simulink library "Lib_Piccolo"  (R2018b)
settings: Solver=VariableStepAuto  StartTime=0.0  StopTime=10.0  RelTol=1e-3
values from neighbouring files (symbols this model uses):
  AccelErrInt2Brakes = 0.15    [SimulationControlConfig16P.m]    (also in SimulationControlConfig16P_LEGACY.m; SimulationControlConfigTAILLESS.m = 0.2; SimulationControlConfigUTAIL.m = 0.2)
  AileronMax = 25    [SimulationControlConfig16P.m]    (also in SimulationControlConfig16P_LEGACY.m; SimulationControlConfigTAILLESS.m; SimulationControlConfigUTAIL.m)
  AileronPower = 0.00268    [SimulationControlConfig16P.m]    (also in SimulationControlConfig16P_LEGACY.m; SimulationControlConfigTAILLESS.m; SimulationControlConfigUTAIL.m)
  AileronSurfaceMax = 45    [SimulationControlConfig16P.m]    (also in SimulationControlConfig16P_LEGACY.m)
  AileronTrim = 0    [SimulationControlConfig16P.m]    (also in SimulationControlConfig16P_LEGACY.m; SimulationControlConfigTAILLESS.m; SimulationControlConfigUTAIL.m)
  Alt = 1000 + TerrainHeight    [SimulationStateConfig.m]
  AltCruise_m = testPlans(testIndx).terrainElevation * 0.3048 + 200    [SimulationControlConfig16P.m]    (also in SimulationControlConfigTAILLESS.m = 1083; SimulationControlConfigUTAIL.m = testPlans(testIndx).terrainElevation * 0.3048 + 152)
  AltitudeRate2PitchCmdIntegratorInit = 0.1    [SimulationControlPre.m]
  AltMax = 10000    [SimulationControlConfig16P.m]    (also in SimulationControlConfig16P_LEGACY.m; SimulationControlConfigTAILLESS.m; SimulationControlConfigUTAIL.m)
  AltMaxAccel = 1.25    [SimulationControlConfig16P.m]    (also in SimulationControlConfig16P_LEGACY.m = 0.9; SimulationControlConfigTAILLESS.m = 1.7; SimulationControlConfigUTAIL.m = 2)
  AltMin = 0    [SimulationControlConfig16P.m]    (also in SimulationControlConfig16P_LEGACY.m; SimulationControlConfigTAILLESS.m; SimulationControlConfigUTAIL.m)
  AltRateCmd2Pitch = 0.50    (= 0.5)    [SimulationControlConfig16P.m]    (also in SimulationControlConfig16P_LEGACY.m = 0.6; SimulationControlConfigTAILLESS.m = 0.2; SimulationControlConfigUTAIL.m = 0.3)
  AltRateError2Pitch = 0.40    (= 0.4)    [SimulationControlConfig16P.m]    (also in SimulationControlConfig16P_LEGACY.m; SimulationControlConfigTAILLESS.m = 0.55; SimulationControlConfigUTAIL.m = 0.55)
  AltRateErrorInt2Pitch = 0.50    (= 0.5)    [SimulationControlConfig16P.m]    (also in SimulationControlConfig16P_LEGACY.m = 0.45; SimulationControlConfigTAILLESS.m; SimulationControlConfigUTAIL.m = 0.75)
  AltRateLpfCutOff = 3    [SimulationControlConfig16P.m]    (also in SimulationControlConfig16P_LEGACY.m; SimulationControlConfigTAILLESS.m = 2; SimulationControlConfigUTAIL.m = 2)
  AutoNosegear2Rudder = 26    [SimulationControlConfig16P.m]    (also in SimulationControlConfig16P_LEGACY.m; SimulationControlConfigTAILLESS.m = 25.2; SimulationControlConfigUTAIL.m = 14)
  b = 5.54    [SimulationControlConfig16P.m]    (also in SimulationControlConfig16P_LEGACY.m; SimulationControlConfigTAILLESS.m = 2.37; SimulationControlConfigUTAIL.m = 2.37)
  Bank2AileronIntegratorInit = 0    [SimulationControlPre.m]
  BankMax_User = BankMax_User/180*pi    (= 0.523598775598)    [SimulationControlConfig16P.m]    (also in SimulationControlConfig16P_LEGACY.m; SimulationControlConfigTAILLESS.m = 0.610865238198; SimulationControlConfigUTAIL.m = 0.628318530718)
  baseLegFlaps = 20    [SimulationControlConfig16P.m]    (also in SimulationControlConfig16P_LEGACY.m = 0; SimulationControlConfigTAILLESS.m = 15; SimulationControlConfigUTAIL.m = 10)
  C = GeneticOpt.C    [SimulationCostFunction.m]
  c = Sw/b    (= 0.841696750903)    [SimulationControlConfig16P.m]    (also in SimulationControlConfig16P_LEGACY.m; SimulationControlConfigTAILLESS.m = 0.354008438819; SimulationControlConfigUTAIL.m = 0.354008438819)
  cell2WheelFactorMG = 5.98    [SimulationSensorConfig16P_LEGACY.m]
  cell2WheelFactorNG = 1    [SimulationSensorConfig16P_LEGACY.m]
  cellSatMaxMG = 15000    [SimulationSensorConfig16P.m]    (also in SimulationSensorConfig16P_LEGACY.m; SimulationSensorConfigTAILLESS7P.m; SimulationSensorConfigUTAIL7P.m)
  cellSatMaxNG = 1000    [SimulationSensorConfig16P.m]    (also in SimulationSensorConfig16P_LEGACY.m; SimulationSensorConfigTAILLESS7P.m; SimulationSensorConfigUTAIL7P.m)
  cellSatMinMG = -15000    [SimulationSensorConfig16P.m]    (also in SimulationSensorConfig16P_LEGACY.m; SimulationSensorConfigTAILLESS7P.m; SimulationSensorConfigUTAIL7P.m)
  cellSatMinNG = -1000    [SimulationSensorConfig16P.m]    (also in SimulationSensorConfig16P_LEGACY.m; SimulationSensorConfigTAILLESS7P.m; SimulationSensorConfigUTAIL7P.m)
  CL_Limit = CL_Max    (= 0.54)    [SimulationControlConfig16P.m]    (also in SimulationControlConfig16P_LEGACY.m; SimulationControlConfigTAILLESS.m; SimulationControlConfigUTAIL.m = 0.53)
  CL_Max = 0.54    [SimulationControlConfig16P.m]    (also in SimulationControlConfig16P_LEGACY.m; SimulationControlConfigTAILLESS.m; SimulationControlConfigUTAIL.m = 0.53)
  CL_Max_Nom = 0.465    [SimulationControlConfig16P.m]    (also in SimulationControlConfig16P_LEGACY.m; SimulationControlConfigTAILLESS.m = 0.39; SimulationControlConfigUTAIL.m)
  CL_Min = 0    [SimulationControlConfig16P.m]    (also in SimulationControlConfig16P_LEGACY.m; SimulationControlConfigTAILLESS.m; SimulationControlConfigUTAIL.m)
  ClimbMaxFraction = 0.35    [SimulationControlConfig16P.m]    (also in SimulationControlConfig16P_LEGACY.m = 0.24; SimulationControlConfigTAILLESS.m = 0.19; SimulationControlConfigUTAIL.m = 0.21)
  ClimboutMaxBank = 7.0    (= 7)    [SimulationControlConfig16P.m]    (also in SimulationControlConfig16P_LEGACY.m; SimulationControlConfigTAILLESS.m = 5; SimulationControlConfigUTAIL.m)
  ClimboutTimer = 7.0    (= 7)    [SimulationControlConfig16P.m]    (also in SimulationControlConfig16P_LEGACY.m; SimulationControlConfigTAILLESS.m; SimulationControlConfigUTAIL.m)
  dCl_per_dFlap = 0.005581818    [SimulationControlConfig16P.m]    (also in SimulationControlConfig16P_LEGACY.m = 0; SimulationControlConfigTAILLESS.m = 0; SimulationControlConfigUTAIL.m = 0)
  DecelerationCmd = 3.1    [SimulationControlConfig16P.m]    (also in SimulationControlConfig16P_LEGACY.m; SimulationControlConfigTAILLESS.m = 0.1; SimulationControlConfigUTAIL.m = 0.1)
  DeRotateLogicEndTimer = abs((NoseDownLimit_Deg-1)/DeRotateRamp_Dps)    [SimulationControlConfig16P.m]    (also in SimulationControlConfig16P_LEGACY.m; SimulationControlConfigTAILLESS.m; SimulationControlConfigUTAIL.m)
  DeRotateLogicHoldNoseUpTimer = 0.1    [SimulationControlConfig16P.m]    (also in SimulationControlConfig16P_LEGACY.m; SimulationControlConfigTAILLESS.m; SimulationControlConfigUTAIL.m)
  DeRotateLogicTimerTimeout = 2    [SimulationControlConfig16P.m]    (also in SimulationControlConfig16P_LEGACY.m; SimulationControlConfigTAILLESS.m; SimulationControlConfigUTAIL.m)
  DeRotateLowerCmdSaturation = 0    [SimulationControlConfig16P.m]    (also in SimulationControlConfig16P_LEGACY.m; SimulationControlConfigTAILLESS.m; SimulationControlConfigUTAIL.m)
  DeRotateRamp_Dps = 3    [SimulationControlConfig16P.m]    (also in SimulationControlConfig16P_LEGACY.m; SimulationControlConfigTAILLESS.m = 8; SimulationControlConfigUTAIL.m = 8)
  DeRotateUpperCmdSaturation = 7    [SimulationControlConfig16P.m]    (also in SimulationControlConfig16P_LEGACY.m; SimulationControlConfigTAILLESS.m; SimulationControlConfigUTAIL.m)
  DescentMaxFraction = 0.22    [SimulationControlConfig16P.m]    (also in SimulationControlConfig16P_LEGACY.m = 0.2; SimulationControlConfigTAILLESS.m = 0.17; SimulationControlConfigUTAIL.m = 0.17)
  DesktopSimTerrainOffset_m = 0.406    [SimulationAircraftConfig.m]
  downwindFlaps = 0    [SimulationControlConfig16P.m]    (also in SimulationControlConfig16P_LEGACY.m; SimulationControlConfigTAILLESS.m; SimulationControlConfigUTAIL.m)
  DP_init = 0.5*1.225*V_init^2    [SimulationControlConfig16P.m]    (also in SimulationControlConfig16P_LEGACY.m; SimulationControlConfigTAILLESS.m; SimulationControlConfigUTAIL.m)
  dscNoiseMG = 1    [SimulationSensorConfig16P_LEGACY.m]
  dscNoiseNG = 0.25    [SimulationSensorConfig16P_LEGACY.m]
  DSCnumBits = 24    [SimulationSensorConfig16P.m]    (also in SimulationSensorConfig16P_LEGACY.m; SimulationSensorConfigTAILLESS7P.m; SimulationSensorConfigUTAIL7P.m)
  DSCRangeMaxMG = 15000    [SimulationSensorConfig16P.m]    (also in SimulationSensorConfig16P_LEGACY.m; SimulationSensorConfigTAILLESS7P.m; SimulationSensorConfigUTAIL7P.m)
  DSCRangeMaxNG = 1000    [SimulationSensorConfig16P.m]    (also in SimulationSensorConfig16P_LEGACY.m; SimulationSensorConfigTAILLESS7P.m; SimulationSensorConfigUTAIL7P.m)
  DSCRangeMinMG = -15000    [SimulationSensorConfig16P.m]    (also in SimulationSensorConfig16P_LEGACY.m; SimulationSensorConfigTAILLESS7P.m; SimulationSensorConfigUTAIL7P.m)
  DSCRangeMinNG = -1000    [SimulationSensorConfig16P.m]    (also in SimulationSensorConfig16P_LEGACY.m; SimulationSensorConfigTAILLESS7P.m; SimulationSensorConfigUTAIL7P.m)
  dt = DLLSim.dt    [SimulationTimeStep.m]    (also in SimulationTrim.m = 0.02)
  EarlyTouchdownThreshold = 3.0    (= 3)    [SimulationControlConfig16P.m]    (also in SimulationControlConfig16P_LEGACY.m; SimulationControlConfigTAILLESS.m = 2.2; SimulationControlConfigUTAIL.m = 2.5)
  ElevatorDeflectionRate = 15    [SimulationControlConfig16P.m]    (also in SimulationControlConfig16P_LEGACY.m = 12; SimulationControlConfigTAILLESS.m = 10; SimulationControlConfigUTAIL.m = 12)
  ElevatorMax = 25    [SimulationControlConfig16P.m]    (also in SimulationControlConfig16P_LEGACY.m; SimulationControlConfigTAILLESS.m; SimulationControlConfigUTAIL.m)
  ElevatorPower = -0.002209    [SimulationControlConfig16P.m]    (also in SimulationControlConfig16P_LEGACY.m; SimulationControlConfigTAILLESS.m = -0.002956; SimulationControlConfigUTAIL.m = -0.00205983)
  ElevatorTrim = -3.5    [SimulationControlConfig16P.m]    (also in SimulationControlConfig16P_LEGACY.m; SimulationControlConfigTAILLESS.m = -6; SimulationControlConfigUTAIL.m = -8)
  elevonBias = 0    [SimulationControlConfig16P.m]    (also in SimulationControlConfig16P_LEGACY.m; SimulationControlConfigTAILLESS.m; SimulationControlConfigUTAIL.m)
  Enable_TAS_Protection = 0    [SimulationControlConfig16P.m]    (also in SimulationControlConfig16P_LEGACY.m; SimulationControlConfigTAILLESS.m; SimulationControlConfigUTAIL.m)
  EnableCrossTrackAbort = 1    [SimulationControlConfig16P.m]    (also in SimulationControlConfigTAILLESS.m; SimulationControlConfigUTAIL.m)
  EnergyBandwidth = 0.02    [SimulationControlConfig16P.m]    (also in SimulationControlConfig16P_LEGACY.m; SimulationControlConfigTAILLESS.m = 0.06; SimulationControlConfigUTAIL.m = 0.06)
  EngineLhFuelCut = 0    [SimulationAircraftConfig.m]
  EngineRhFuelCut = 0    [SimulationAircraftConfig.m]
  FastThrottleRate = 0.075    [SimulationControlConfig16P.m]    (also in SimulationControlConfig16P_LEGACY.m = 0.05; SimulationControlConfigTAILLESS.m = 0.1; SimulationControlConfigUTAIL.m = 0.1)
  FilterWarmUpTime = 2    [SimulationSensorConfig16P.m]    (also in SimulationSensorConfig16P_LEGACY.m; SimulationSensorConfigTAILLESS7P.m; SimulationSensorConfigUTAIL7P.m)
  finalApproachFlaps = 20    [SimulationControlConfig16P.m]    (also in SimulationControlConfig16P_LEGACY.m = 0; SimulationControlConfigTAILLESS.m = 22; SimulationControlConfigUTAIL.m = 10)
  FinalDescentSlope_Deg = testPlans(testIndx).descentSlope    [SimulationControlConfig16P.m]    (also in SimulationControlConfig16P_LEGACY.m; SimulationControlConfigTAILLESS.m; SimulationControlConfigUTAIL.m)
  flapMax = 0    [SimulationControlConfig16P.m]    (also in SimulationControlConfig16P_LEGACY.m; SimulationControlConfigTAILLESS.m; SimulationControlConfigUTAIL.m)
  flapRate = 7.5    [SimulationControlConfig16P.m]    (also in SimulationControlConfig16P_LEGACY.m; SimulationControlConfigTAILLESS.m = 6.6; SimulationControlConfigUTAIL.m)
  FlareHeight = 5    [SimulationControlConfig16P.m]    (also in SimulationControlConfig16P_LEGACY.m = 4.8; SimulationControlConfigTAILLESS.m = 2.5; SimulationControlConfigUTAIL.m = 2)
  FlareVerticalRate_mps = -0.4    [SimulationControlConfig16P.m]    (also in SimulationControlConfig16P_LEGACY.m = -0.5; SimulationControlConfigTAILLESS.m = -0.15; SimulationControlConfigUTAIL.m = -0.15)
  Fp_Aileron = 0.55*2*pi*RollRateLpfCutoff*dt    [SimulationControlConfig16P.m]    (also in SimulationControlConfig16P_LEGACY.m; SimulationControlConfigTAILLESS.m; SimulationControlConfigUTAIL.m)
  Fp_Alt = 0.55*AltBandwidth    (= 0.099)    [SimulationControlConfig16P.m]    (also in SimulationControlConfig16P_LEGACY.m; SimulationControlConfigTAILLESS.m = 0.587477826221; SimulationControlConfigUTAIL.m = 0.69115038379)
  Fp_AltRate = 0.55*2*pi*AltRateLpfCutOff*dt    [SimulationControlConfig16P.m]    (also in SimulationControlConfig16P_LEGACY.m; SimulationControlConfigTAILLESS.m; SimulationControlConfigUTAIL.m)
  Fp_Elevator = 0.55*2*pi*PitchRateLpfCutoff*dt    [SimulationControlConfig16P.m]    (also in SimulationControlConfig16P_LEGACY.m; SimulationControlConfigTAILLESS.m; SimulationControlConfigUTAIL.m)
  Fp_Energy = 0.55*2*pi*EnergyBandwidth    (= 0.069115038379)    [SimulationControlConfig16P.m]    (also in SimulationControlConfig16P_LEGACY.m; SimulationControlConfigTAILLESS.m = 0.207345115137; SimulationControlConfigUTAIL.m = 0.207345115137)
  Fp_Energy2 = 0.55*2*pi*EnergyBandwidth*dt    [SimulationControlConfig16P.m]    (also in SimulationControlConfig16P_LEGACY.m; SimulationControlConfigTAILLESS.m; SimulationControlConfigUTAIL.m)
  Fp_Pitch = 0.55*2*pi*PitchBandwidth    (= 2.76460153516)    [SimulationControlConfig16P.m]    (also in SimulationControlConfig16P_LEGACY.m = 3.11017672705; SimulationControlConfigTAILLESS.m = 3.80132711084; SimulationControlConfigUTAIL.m = 2.41902634326)
  Fp_Pitch_2 = 0.55*2*pi*PitchBandwidth*dt    [SimulationControlConfig16P.m]    (also in SimulationControlConfig16P_LEGACY.m; SimulationControlConfigTAILLESS.m; SimulationControlConfigUTAIL.m)
  Fp_Roll = RollBandwidth^2    (= 1)    [SimulationControlConfig16P.m]    (also in SimulationControlConfig16P_LEGACY.m = 1.44; SimulationControlConfigTAILLESS.m; SimulationControlConfigUTAIL.m)
  Fp_Rudder = 0.55*2*pi*YawRateLpfCutoff*dt    [SimulationControlConfig16P.m]    (also in SimulationControlConfig16P_LEGACY.m; SimulationControlConfigTAILLESS.m; SimulationControlConfigUTAIL.m)
  Fp_TAS = 0.55*2*pi*TASBandwidth    (= 0.103672557568)    [SimulationControlConfig16P.m]    (also in SimulationControlConfig16P_LEGACY.m; SimulationControlConfigTAILLESS.m = 0.172787595947; SimulationControlConfigUTAIL.m = 0.172787595947)
  Fp_TAS_Filter = 2*pi*TasLpfCutoff*dt    [SimulationControlConfig16P.m]    (also in SimulationControlConfig16P_LEGACY.m; SimulationControlConfigTAILLESS.m; SimulationControlConfigUTAIL.m)
  Fp_Turn = 0.55*2*pi*TurnErrLPFcutoff    (= 0.0345575191895)    [SimulationControlConfig16P.m]    (also in SimulationControlConfig16P_LEGACY.m; SimulationControlConfigTAILLESS.m = 0.172787595947; SimulationControlConfigUTAIL.m = 0.172787595947)
  Fp_TurnDerr = 0.55*2*pi*TurnDerivativeLPFcutoff    (= 0.0345575191895)    [SimulationControlConfig16P.m]    (also in SimulationControlConfig16P_LEGACY.m; SimulationControlConfigTAILLESS.m = 0.172787595947; SimulationControlConfigUTAIL.m = 0.172787595947)
  FTV = 3    [SimulationAircraftConfig.m]
  ftvStaticPositionError = 1/1.18    (= 0.847457627119)    [SimulationSensorConfig16P.m]    (also in SimulationSensorConfig16P_LEGACY.m; SimulationSensorConfigTAILLESS7P.m = 1; SimulationSensorConfigUTAIL7P.m = 1)
  g = 9.81    [SimulationStateConfig.m]
  GustSpd_Kts = testPlans(testIndx).gustSpd    [SimulationStateConfig.m]
  GustTriggerVal = testPlans(testIndx).gustTriggerVal    [SimulationStateConfig.m]
  HeadingErr2TurnRate = 0.5    [SimulationControlConfig16P.m]    (also in SimulationControlConfig16P_LEGACY.m; SimulationControlConfigTAILLESS.m; SimulationControlConfigUTAIL.m)
  HeadingErrDer2TurnRate = 0.3    [SimulationControlConfig16P.m]    (also in SimulationControlConfig16P_LEGACY.m; SimulationControlConfigTAILLESS.m; SimulationControlConfigUTAIL.m)
  IASbounce = IASstall*0.8    [SimulationControlPre.m]
  IAScruiseCMD = sqrt(2*m*9.81/(1.225*Sw*CL_cruise))    [SimulationControlConfig16P.m]    (also in SimulationControlConfig16P_LEGACY.m; SimulationControlConfigTAILLESS.m; SimulationControlConfigUTAIL.m)
  IASfinalCMD = 1.12 * IASmin    [SimulationControlConfig16P.m]    (also in SimulationControlConfig16P_LEGACY.m = 1.10 * IASmin; SimulationControlConfigTAILLESS.m = 1.10 * IASmin; SimulationControlConfigUTAIL.m = 1.15 * IASmin)
  IASflareCMD = IASstall    [SimulationControlConfig16P.m]    (also in SimulationControlConfig16P_LEGACY.m; SimulationControlConfigTAILLESS.m; SimulationControlConfigUTAIL.m)
  IASmax = 64    [SimulationControlConfig16P.m]    (also in SimulationControlConfig16P_LEGACY.m = 46; SimulationControlConfigTAILLESS.m = 38.58; SimulationControlConfigUTAIL.m = 35)
  IASmin = sqrt(2*m*9.81/(1.225*Sw*0.9*CL_Max_Nom))    [SimulationControlConfig16P.m]    (also in SimulationControlConfig16P_LEGACY.m; SimulationControlConfigTAILLESS.m; SimulationControlConfigUTAIL.m)
  IASshortCMD = IASstall    [SimulationControlConfig16P.m]    (also in SimulationControlConfig16P_LEGACY.m; SimulationControlConfigTAILLESS.m; SimulationControlConfigUTAIL.m)
  IASstall = sqrt(2*m*9.81/(1.225*Sw*CL_Max))    [SimulationControlConfig16P.m]    (also in SimulationControlConfig16P_LEGACY.m; SimulationControlConfigTAILLESS.m; SimulationControlConfigUTAIL.m)
  inFlight = 1    [SimulationControlConfig16P.m]    (also in SimulationControlConfigTAILLESS.m; SimulationControlConfigUTAIL.m)
  JetCatOffset = 5    [SimulationControlConfig16P.m]    (also in SimulationControlConfig16P_LEGACY.m)
  LaunchRollingElevator = -1.5    [SimulationControlConfig16P.m]    (also in SimulationControlConfig16P_LEGACY.m; SimulationControlConfigTAILLESS.m = 1; SimulationControlConfigUTAIL.m = 1)
  ldg_NosegearMax = 10    [SimulationControlConfig16P.m]    (also in SimulationControlConfig16P_LEGACY.m; SimulationControlConfigTAILLESS.m; SimulationControlConfigUTAIL.m)
  ldg_TrackVyErrInt2Nosegear = 0.1250    (= 0.125)    [SimulationControlConfig16P.m]    (also in SimulationControlConfig16P_LEGACY.m; SimulationControlConfigTAILLESS.m = 0.00714285714286; SimulationControlConfigUTAIL.m = 0.00714285714286)
  ldg_TrackVyErrPro2Nosegear = 0.35    [SimulationControlConfig16P.m]    (also in SimulationControlConfig16P_LEGACY.m; SimulationControlConfigTAILLESS.m = 0.0546666666667; SimulationControlConfigUTAIL.m = 0.0546666666667)
  ldg_TrackY2Vy = 0.07    [SimulationControlConfig16P.m]    (also in SimulationControlConfig16P_LEGACY.m; SimulationControlConfigTAILLESS.m = 0.17; SimulationControlConfigUTAIL.m = 0.17)
  ldg_Vy2NosegearScalingPower = 1.075    [SimulationControlConfig16P.m]    (also in SimulationControlConfig16P_LEGACY.m; SimulationControlConfigTAILLESS.m = 0.6; SimulationControlConfigUTAIL.m = 0.5)
  ldg_Y2VyScalingPower = 0.175    [SimulationControlConfig16P.m]    (also in SimulationControlConfig16P_LEGACY.m; SimulationControlConfigTAILLESS.m = 0; SimulationControlConfigUTAIL.m = 0)
  ldg_YawRate2Nosegear = 0.175    [SimulationControlConfig16P.m]    (also in SimulationControlConfig16P_LEGACY.m; SimulationControlConfigTAILLESS.m = 0.065; SimulationControlConfigUTAIL.m = 0.065)
  LiftSlope = 0.064285    [SimulationControlConfig16P.m]    (also in SimulationControlConfig16P_LEGACY.m; SimulationControlConfigTAILLESS.m = 0.058631; SimulationControlConfigUTAIL.m)
  LPFaileronInit = 0    [SimulationControlPre.m]
  LPFclestInit = 0    [SimulationControlPre.m]
  LPFenergyFFInit = 0    [SimulationControlPre.m]
  LPFtasInit = V_init + 2    [SimulationControlPre.m]
  LPFthrottleInit = ThrottleTrim    [SimulationControlPre.m]
  LPFturnErrInit = 0    [SimulationControlPre.m]
  ... (+115 more)
undefined symbols (not defined in the file or in its folder): abortFlag, alphaHPF, apmDelay, BRWNOUT, CRAWOR, CRAWUR, DiscIntNeverNeededParam, DLLSim, DLLSimStep, ECOMOR, ECOMUR, Fp_Tas, GustTrigger_HeightAgl_m, IPSTAT, LCINTEG, Ldg_Persist_Time, LOWER_FLAGS, MSG_ENABLE, NoiseStd, OLDVAL, OVERRIDE_ENABLE, OVERRIDE_VALUE, REBOOT, reversionEnable, revIASMax, revIASMin, revPitchMax, revPitchMin, revPitchRateMax, revRollMax, revRollRateMax, SAMPLE, SCALON, SensorModel, sigbuilder_block, Sim_Vx, Sim_Vy, Sim_Vz, Sim_Xpos, Sim_Ypos, Sim_Zpos, SYSOR, SYSUR, TARE, TEMPOR, TEMPUR, testIndx, testPlan, testPlans, Trim_piccoloInCmd, Trim_REFSI_FD_IN_nmodeCgShifterCmd_Ft, Trim_REFSI_FD_IN_nmodeFlapLhIBCmd_Deg, Trim_REFSI_FD_IN_nmodeFlapLhOBCmd_Deg, Trim_REFSI_FD_IN_nmodeFlapRhIBCmd_Deg, Trim_REFSI_FD_IN_nmodeFlapRhOBCmd_Deg, Trim_REFSI_FD_IN_nmodeSlatLhCmd_Deg, Trim_REFSI_FD_IN_nmodeSlatRhCmd_Deg, Trim_REFSI_FD_IN_nmodeSplrLhInbdCmd_Deg, Trim_REFSI_FD_IN_nmodeSplrLhOutbdCmd_Deg ... (+5)
libraries: simulink x866, aerolibconvert2 x60, $bdroot x52, aerolibatmos2 x5, dspswit3 x5, simulink_extras x4, dsparch4 x2, Lib_Piccolo_Alt x2, eeGeneralControl x1, dspindex x1
(part 44 of 44)

== system Lib_Piccolo/Ground Detection Systems/WoW Wrapper/Variant Subsystem/Load Cell WoW Model 20/WOW Module/Subsystem/Health Check/NG DSC Fail Logic/NG Data Validation ==
  AP Mode : Inport
  WOW_N : Inport  Port=2
  AND : Logic  IconShape=distinctive  AllPortsSameDT=off  OutDataTypeStr=boolean
  AND1 : Logic  IconShape=distinctive  AllPortsSameDT=off  OutDataTypeStr=boolean
  Abs : Abs
  Compare To Constant : simulink/Logic and Bit Operations/Compare To Constant  relop=>  const=SensorModel.WOW.Cell.satMaxNGWheel  OutDataTypeStr=boolean
  Compare To Constant1 : simulink/Logic and Bit Operations/Compare To Constant  relop=<  const=SensorModel.WOW.Cell.satMinNGWheel  OutDataTypeStr=boolean
  Compare To Constant2 : simulink/Logic and Bit Operations/Compare To Constant  relop=>  const=SensorModel.WOW.Cell.loadThresholdLower_N  OutDataTypeStr=boolean
  Greater Than Climbout : simulink/Logic and Bit Operations/Compare To Constant  relop=>  const=3  OutDataTypeStr=boolean
  Is on Final : simulink/Logic and Bit Operations/Compare To Constant  relop===  const=8  OutDataTypeStr=boolean
  Less Than Final Mode : simulink/Logic and Bit Operations/Compare To Constant  relop=<  const=8  OutDataTypeStr=boolean
  OR : Logic  Operator=OR  IconShape=distinctive  AllPortsSameDT=off  OutDataTypeStr=boolean
  OR1 : Logic  IconShape=distinctive  AllPortsSameDT=off  OutDataTypeStr=boolean
  Persistence Counter : Subsystem
  Persistence Counter1 : $bdroot/Ground Detection Systems/WoW Wrapper/Variant Subsystem/Load Cell WoW Model 20/WOW Module/Subsystem/Health Check/MGR DSC Fail Logic/MG Data Validation/Persistence Counter  SystemSampleTime=-1
  Persistence Counter2 : $bdroot/Ground Detection Systems/WoW Wrapper/Variant Subsystem/Load Cell WoW Model 20/WOW Module/Subsystem/Health Check/MGR DSC Fail Logic/MG Data Validation/Persistence Counter  SystemSampleTime=-1
  INVALID : Outport
  IN_FLIGHT_BIAS : Outport  Port=2
  FINAL_BIAS : Outport  Port=3
  wires:
  WOW_N/1 -> Compare To Constant/1, Abs/1, Compare To Constant1/1
  Compare To Constant/1 -> OR/1
  Compare To Constant1/1 -> OR/2
  OR/1 -> Persistence Counter/1(Trigger/!Rst)
  Persistence Counter/1(TIMEOUT) -> INVALID/1
  Persistence Counter1/1 -> IN_FLIGHT_BIAS/1
  AP Mode/1 -> Is on Final/1, Greater Than Climbout/1, Less Than Final Mode/1
  Compare To Constant2/1 -> AND1/2, AND/2
  AND/1 -> Persistence Counter1/1
  OR1/1 -> AND/1
  Less Than Final Mode/1 -> OR1/2
  Greater Than Climbout/1 -> OR1/1
  Persistence Counter2/1 -> FINAL_BIAS/1
  AND1/1 -> Persistence Counter2/1
  Is on Final/1 -> AND1/1
  Abs/1 -> Compare To Constant2/1

== system Lib_Piccolo/Ground Detection Systems/WoW Wrapper/Variant Subsystem/Load Cell WoW Model 20/WOW Module/Subsystem/Health Check/MGR DSC Fail Logic/MG Data Validation/Persistence Counter ==
  Trigger/!Rst : Inport  OutDataTypeStr=boolean
  Compare To Constant : simulink/Logic and Bit Operations/Compare To Constant  relop=>=  const=SensorModel.WOW.Cell.INVALID_COUNTS  OutDataTypeStr=boolean
  Counter : dspswit3/Counter  Direction=Up  CountEvent=Non-zero sample  CounterSize=8 bits  MaxCount=10  InitialCount=0  Output=Count  HitValue=32  ResetInput=on  SamplesPerFrame=1  Ts=1  CntDtype=uint8  HitDtype=Logical
  Limit Count : $bdroot/Ground Detection Systems/WoW Wrapper/Variant Subsystem/Load Cell WoW Model 20/WOW Module/Subsystem/Comms Timeout Logic/LOAD Timeout Counter/Limit Count  SystemSampleTime=-1
  NOT : Logic  Operator=NOT  IconShape=distinctive  AllPortsSameDT=off  OutDataTypeStr=boolean
  TIMEOUT : Outport
  wires:
  Counter/1 -> Compare To Constant/1
  NOT/1 -> Counter/2
  Trigger/!Rst/1 -> Limit Count/2, NOT/1
  Compare To Constant/1 -> TIMEOUT/1, Limit Count/1
  Limit Count/1 -> Counter/1

== system Lib_Piccolo/Ground Detection Systems/WoW Wrapper/Variant Subsystem/Load Cell WoW Model 20/WOW Module/Subsystem/Health Check/NG DSC Fail Logic/NG Data Validation/Persistence Counter ==
  Trigger/!Rst : Inport  OutDataTypeStr=boolean
  Compare To Constant : simulink/Logic and Bit Operations/Compare To Constant  relop=>=  const=SensorModel.WOW.Cell.INVALID_COUNTS  OutDataTypeStr=boolean
  Counter : dspswit3/Counter  Direction=Up  CountEvent=Non-zero sample  CounterSize=8 bits  MaxCount=10  InitialCount=0  Output=Count  HitValue=32  ResetInput=on  SamplesPerFrame=1  Ts=1  CntDtype=uint8  HitDtype=Logical
  Limit Count : $bdroot/Ground Detection Systems/WoW Wrapper/Variant Subsystem/Load Cell WoW Model 20/WOW Module/Subsystem/Comms Timeout Logic/LOAD Timeout Counter/Limit Count  SystemSampleTime=-1
  NOT : Logic  Operator=NOT  IconShape=distinctive  AllPortsSameDT=off  OutDataTypeStr=boolean
  TIMEOUT : Outport
  wires:
  Counter/1 -> Compare To Constant/1
  NOT/1 -> Counter/2
  Trigger/!Rst/1 -> Limit Count/2, NOT/1
  Compare To Constant/1 -> TIMEOUT/1, Limit Count/1
  Limit Count/1 -> Counter/1

== matlab function Lib_Piccolo/Control Allocation/M8 Flap-to-Drag/Surface Mixing Function ==
  data: Pic_AileronCmd input; PrtAileronUpperCmd output; Pic_ElevatorCmd input; PrtAileronLowerCmd output; StbdAileronUpperCmd output; StbdAileronLowerCmd output; PrtInbElevonCmd output; StbdInbdElevonCmd output; PrtOutElevonCmd output; StbdOutdElevonCmd output; ElevatorUtailCmd output; AftFlapCmd output; Pic_RudderCmd input; PylonRudderCmd output; WingletRudderCmd output; UTailRudderCmd output; Pic_FlapCmd input
function [PrtAileronUpperCmd, PrtAileronLowerCmd, StbdAileronUpperCmd, StbdAileronLowerCmd,...
          PrtInbElevonCmd, StbdInbdElevonCmd, PrtOutElevonCmd, StbdOutdElevonCmd,...
          ElevatorUtailCmd, AftFlapCmd,...
          PylonRudderCmd, WingletRudderCmd, UTailRudderCmd]= fcn(Pic_AileronCmd, Pic_ElevatorCmd, Pic_RudderCmd, Pic_FlapCmd)

      % Mixing flap commands to split ailerons
      PrtAileronUpperCmd = max(-1 * Pic_FlapCmd + Pic_AileronCmd, -45);
      PrtAileronLowerCmd =  min(Pic_FlapCmd + Pic_AileronCmd, 45);

      StbdAileronUpperCmd = min(Pic_FlapCmd + Pic_AileronCmd, 45);
      StbdAileronLowerCmd =  max(-1 * Pic_FlapCmd + Pic_AileronCmd, -45);
          
      % Pitch and Roll mixed to Elevons
      PrtInbElevonCmd   = max(Pic_AileronCmd + Pic_ElevatorCmd);
      StbdInbdElevonCmd = max((-1)*Pic_AileronCmd + Pic_ElevatorCmd);
      
      PrtOutElevonCmd   = max(Pic_AileronCmd + Pic_ElevatorCmd);
      StbdOutdElevonCmd = max((-1)*Pic_AileronCmd + Pic_ElevatorCmd);
      
      ElevatorUtailCmd = 0;
      AftFlapCmd = Pic_ElevatorCmd; 
      
      PylonRudderCmd   = Pic_RudderCmd;
      
      WingletRudderCmd = Pic_RudderCmd;
            
      UTailRudderCmd   = 0;      
end

== matlab function Lib_Piccolo/Throttle Control (Alt Mode)/Filter and Throttle Cut/LPF Throttle Alpha/LPF Alpha Throttle ==
  data: xFiltOld input; dt input; xNew input; bandwidth input; xFilt output
function xFilt = fcn(xFiltOld ,dt, xNew, bandwidth)
% Piccolo FWG 3 1st order IIR Lowpass filter
alpha = dt*2*pi*bandwidth*abs(xNew-xFiltOld)/0.1;
if(alpha<1.0)
    xFilt =xNew * alpha + xFiltOld*(1-alpha);
else
    xFilt=xNew;
end

== matlab function Lib_Piccolo/Control Allocation/M2/Surface Mixing Function ==
  data: Pic_AileronCmd input; PrtAileronUpperCmd output; Pic_ElevatorCmd input; PrtAileronLowerCmd output; StbdAileronUpperCmd output; StbdAileronLowerCmd output; PrtInbElevonCmd output; StbdInbdElevonCmd output; PrtOutElevonCmd output; StbdOutdElevonCmd output; ElevatorUtailCmd output; AftFlapCmd output; Pic_RudderCmd input; PylonRudderCmd output; WingletRudderCmd output; UTailRudderCmd output; Pic_FlapCmd input; elevonBias input
function [PrtAileronUpperCmd, PrtAileronLowerCmd, StbdAileronUpperCmd, StbdAileronLowerCmd,...
          PrtInbElevonCmd, StbdInbdElevonCmd, PrtOutElevonCmd, StbdOutdElevonCmd,...
          ElevatorUtailCmd, AftFlapCmd,...
          PylonRudderCmd, WingletRudderCmd, UTailRudderCmd]= fcn(Pic_AileronCmd, Pic_ElevatorCmd, Pic_RudderCmd, Pic_FlapCmd, elevonBias)

      PrtAileronUpperCmd = Pic_AileronCmd;
      PrtAileronLowerCmd = Pic_AileronCmd;
      
      StbdAileronUpperCmd = Pic_AileronCmd;
      StbdAileronLowerCmd = Pic_AileronCmd;
       
      PrtInbElevonCmd   = Pic_AileronCmd;
      StbdInbdElevonCmd = Pic_AileronCmd;
      
      PrtOutElevonCmd   = PrtInbElevonCmd;
      StbdOutdElevonCmd = StbdInbdElevonCmd;
      
      % Bias elevons on flap deployment
      if(Pic_FlapCmd > 15.5)
        PrtInbElevonCmd = PrtInbElevonCmd + elevonBias; 
        PrtOutElevonCmd = PrtOutElevonCmd + elevonBias;
        
        StbdInbdElevonCmd = StbdInbdElevonCmd - elevonBias;
        StbdOutdElevonCmd = StbdOutdElevonCmd - elevonBias;
      end
      
      ElevatorUtailCmd = Pic_ElevatorCmd;
      AftFlapCmd = Pic_ElevatorCmd; 
      
      PylonRudderCmd   = Pic_RudderCmd;
      
      WingletRudderCmd = Pic_RudderCmd;
      
      UTailRudderCmd   = Pic_RudderCmd;      
end

== matlab function Lib_Piccolo/Throttle Control (Airspeed Mode)/Subsystem/LPF Throttle Alpha/LPF Alpha Throttle ==
  data: xFiltOld input; dt input; xNew input; bandwidth input; xFilt output
function xFilt = fcn(xFiltOld ,dt, xNew, bandwidth)
% Piccolo FWG 3 1st order IIR Lowpass filter
alpha = dt*2*pi*bandwidth*abs(xNew-xFiltOld)/0.1;
if(alpha<1.0)
    xFilt =xNew * alpha + xFiltOld*(1-alpha);
else
    xFilt=xNew;
end

== matlab function Lib_Piccolo/Control Allocation/M7/Surface Mixing Function ==
  data: Pic_AileronCmd input; PrtAileronUpperCmd output; Pic_ElevatorCmd input; PrtAileronLowerCmd output; StbdAileronUpperCmd output; StbdAileronLowerCmd output; PrtInbElevonCmd output; StbdInbdElevonCmd output; PrtOutElevonCmd output; StbdOutdElevonCmd output; ElevatorUtailCmd output; AftFlapCmd output; Pic_RudderCmd input; PylonRudderCmd output; WingletRudderCmd output; UTailRudderCmd output
function [PrtAileronUpperCmd, PrtAileronLowerCmd, StbdAileronUpperCmd, StbdAileronLowerCmd,...
          PrtInbElevonCmd, StbdInbdElevonCmd, PrtOutElevonCmd, StbdOutdElevonCmd,...
          ElevatorUtailCmd, AftFlapCmd,...
          PylonRudderCmd, WingletRudderCmd, UTailRudderCmd]= fcn(Pic_AileronCmd, Pic_ElevatorCmd, Pic_RudderCmd)

      PrtAileronUpperCmd = Pic_AileronCmd;
      PrtAileronLowerCmd = Pic_AileronCmd;
      
      StbdAileronUpperCmd = (-1)*Pic_AileronCmd;
      StbdAileronLowerCmd = (-1)*Pic_AileronCmd;
      
      PrtInbElevonCmd   = max(Pic_AileronCmd + Pic_ElevatorCmd);
      StbdInbdElevonCmd = max((-1)*Pic_AileronCmd + Pic_ElevatorCmd);
      
      PrtOutElevonCmd   = max(Pic_AileronCmd + Pic_ElevatorCmd);
      StbdOutdElevonCmd = max((-1)*Pic_AileronCmd + Pic_ElevatorCmd);
      
      ElevatorUtailCmd = Pic_ElevatorCmd;
      AftFlapCmd = Pic_ElevatorCmd; 
      
      PylonRudderCmd   = Pic_RudderCmd;
      
      WingletRudderCmd = Pic_RudderCmd;
       
      UTailRudderCmd   = Pic_RudderCmd;      
end

== matlab function Lib_Piccolo/Control Allocation/M8/Surface Mixing Function ==
  data: Pic_AileronCmd input; PrtAileronUpperCmd output; Pic_ElevatorCmd input; PrtAileronLowerCmd output; StbdAileronUpperCmd output; StbdAileronLowerCmd output; PrtInbElevonCmd output; StbdInbdElevonCmd output; PrtOutElevonCmd output; StbdOutdElevonCmd output; ElevatorUtailCmd output; AftFlapCmd output; Pic_RudderCmd input; PylonRudderCmd output; WingletRudderCmd output; UTailRudderCmd output
function [PrtAileronUpperCmd, PrtAileronLowerCmd, StbdAileronUpperCmd, StbdAileronLowerCmd,...
          PrtInbElevonCmd, StbdInbdElevonCmd, PrtOutElevonCmd, StbdOutdElevonCmd,...
          ElevatorUtailCmd, AftFlapCmd,...
          PylonRudderCmd, WingletRudderCmd, UTailRudderCmd]= fcn(Pic_AileronCmd, Pic_ElevatorCmd, Pic_RudderCmd)

      PrtAileronUpperCmd = Pic_AileronCmd;
      PrtAileronLowerCmd = Pic_AileronCmd;
      
      StbdAileronUpperCmd = (-1)*Pic_AileronCmd;
      StbdAileronLowerCmd = (-1)*Pic_AileronCmd;
      
      PrtInbElevonCmd   = max(Pic_AileronCmd + Pic_ElevatorCmd);
      StbdInbdElevonCmd = max((-1)*Pic_AileronCmd + Pic_ElevatorCmd);
      
      PrtOutElevonCmd   = max(Pic_AileronCmd + Pic_ElevatorCmd);
      StbdOutdElevonCmd = max((-1)*Pic_AileronCmd + Pic_ElevatorCmd);
      
      ElevatorUtailCmd = 0;
      AftFlapCmd = Pic_ElevatorCmd; 
      
      PylonRudderCmd   = Pic_RudderCmd;
      
      WingletRudderCmd = Pic_RudderCmd;
            
      UTailRudderCmd   = 0;      
end

== matlab function Lib_Piccolo/A//C Dynamics/Raw Sensor Sources Alternate/MATLAB Function ==
  data: u input; y output
function y = fcn(u)
if u > 180
    y = u-360;
else
    y = u;
end

== matlab function Lib_Piccolo/Throttle Control (Alt Mode)/LPF Energy Alpha/LPF Alpha Energy ==
  data: xFiltOld input; dt input; xNew input; bandwidth input; xFilt output
function xFilt = fcn(xFiltOld ,dt, xNew, bandwidth)
% Piccolo FWG 3 1st order IIR Lowpass filter
alpha = dt*2*pi*bandwidth*abs(xNew-xFiltOld)/0.1;
if(alpha<1.0)
    xFilt =xNew * alpha + xFiltOld*(1-alpha);
else
    xFilt=xNew;
end

== matlab function Lib_Piccolo/Bank to Aileron/Bank Angle Limit Calculation/Load Factors (nMax,nMin) at current conditions  ==
  data: Q input; nMax output; Sw input; CL_Limit input; CL_Min input; m input; nMax_User input; nMin_User input; nMin output
function [nMax, nMin] = fcn(Q, Sw, CL_Limit,CL_Min, m, nMax_User, nMin_User)

nAero_Max=Sw*Q*CL_Limit/(m*9.81);
nAero_Min=Sw*Q*CL_Min/(m*9.81);
nMax=min(nMax_User,nAero_Max);
nMin=max(nMin_User, nAero_Min);
end

== matlab function Lib_Piccolo/Bank to Aileron/Body To Euler Translation ==
  data: p input; PhiDot output; q input; r input; Phi input; Theta input
function PhiDot = fcn(p, q, r, Phi, Theta)
if abs(Theta)/pi*180<50
    PhiDot=p+tan(Theta)*(q*sin(Phi)+r*cos(Phi));
else 
    PhiDot=p;
end

== matlab function Lib_Piccolo/A//C Dynamics Full Interface/Raw Sensor Sources Alternate/MATLAB Function ==
  data: u input; y output
function y = fcn(u)
if u > 180
    y = u-360;
else
    y = u;
end

== matlab function Lib_Piccolo/Control Allocation/M2 Flap-to-Drag /Surface Mixing Function ==
  data: Pic_AileronCmd input; PrtAileronUpperCmd output; Pic_ElevatorCmd input; PrtAileronLowerCmd output; StbdAileronUpperCmd output; StbdAileronLowerCmd output; PrtInbElevonCmd output; StbdInbdElevonCmd output; PrtOutElevonCmd output; StbdOutdElevonCmd output; ElevatorUtailCmd output; AftFlapCmd output; Pic_RudderCmd input; PylonRudderCmd output; WingletRudderCmd output; UTailRudderCmd output; Pic_FlapCmd input; elevonBias input; AileronMax input
function [PrtAileronUpperCmd, PrtAileronLowerCmd, StbdAileronUpperCmd, StbdAileronLowerCmd,...
          PrtInbElevonCmd, StbdInbdElevonCmd, PrtOutElevonCmd, StbdOutdElevonCmd,...
          ElevatorUtailCmd, AftFlapCmd,...
          PylonRudderCmd, WingletRudderCmd, UTailRudderCmd]= fcn(Pic_AileronCmd, Pic_ElevatorCmd, Pic_RudderCmd, Pic_FlapCmd, elevonBias, AileronMax)
    
      %Roll saturation limits
      if(Pic_AileronCmd > AileronMax)
          Pic_AileronCmd = AileronMax;
      elseif(Pic_AileronCmd < -1*AileronMax)
          Pic_AileronCmd = -1*AileronMax;
      end
      
      % If not commanding flaps, mix ailerons together
      if(Pic_FlapCmd < 0.1)
          PrtAileronUpperCmd = Pic_AileronCmd;
          PrtAileronLowerCmd = Pic_AileronCmd;

          StbdAileronUpperCmd = Pic_AileronCmd;
          StbdAileronLowerCmd = Pic_AileronCmd;
          
      % Else, mix to split ailerons
      else
          PrtAileronUpperCmd = -1 * Pic_FlapCmd + Pic_AileronCmd;
          PrtAileronLowerCmd = Pic_FlapCmd + Pic_AileronCmd;
          
          StbdAileronUpperCmd = Pic_FlapCmd + Pic_AileronCmd;
          StbdAileronLowerCmd = -1 * Pic_FlapCmd + Pic_AileronCmd;
          
          %If top or bottom aileron becomes saturated, prioritize roll authority
          if(PrtAileronUpperCmd <= -1*AileronMax)
              PrtAileronLowerCmd = 2*Pic_AileronCmd+AileronMax;
              PrtAileronUpperCmd = -1*AileronMax;
              StbdAileronUpperCmd = PrtAileronLowerCmd;
              StbdAileronLowerCmd = PrtAileronUpperCmd;
          elseif(PrtAileronLowerCmd >= AileronMax)
              PrtAileronUpperCmd = 2*Pic_AileronCmd-AileronMax;
              PrtAileronLowerCmd = AileronMax;
              StbdAileronUpperCmd = PrtAileronLowerCmd;
              StbdAileronLowerCmd = PrtAileronUpperCmd;
          end
      end
      
      PrtInbElevonCmd   = Pic_AileronCmd;
      StbdInbdElevonCmd = Pic_AileronCmd;
      
      PrtOutElevonCmd   = PrtInbElevonCmd;
      StbdOutdElevonCmd = StbdInbdElevonCmd;  
      
      % Bias elevons on split-Aileron deployment
      if(Pic_FlapCmd > 15.5)
        PrtInbElevonCmd = PrtInbElevonCmd + elevonBias; 
        PrtOutElevonCmd = PrtOutElevonCmd + elevonBias;
        
        StbdInbdElevonCmd = StbdInbdElevonCmd - elevonBias;
        StbdOutdElevonCmd = StbdOutdElevonCmd - elevonBias;
      end
        
      ElevatorUtailCmd = Pic_ElevatorCmd;
      AftFlapCmd = Pic_ElevatorCmd; 
      
      PylonRudderCmd   = Pic_RudderCmd;
      
      WingletRudderCmd = Pic_RudderCmd;
      
      UTailRudderCmd   = Pic_RudderCmd;      
end

== matlab function Lib_Piccolo/Control Allocation/M2 Flaperon/Surface Mixing Function ==
  data: Pic_AileronCmd input; PrtAileronUpperCmd output; Pic_ElevatorCmd input; PrtAileronLowerCmd output; StbdAileronUpperCmd output; StbdAileronLowerCmd output; PrtInbElevonCmd output; StbdInbdElevonCmd output; PrtOutElevonCmd output; StbdOutdElevonCmd output; ElevatorUtailCmd output; AftFlapCmd output; Pic_RudderCmd input; PylonRudderCmd output; WingletRudderCmd output; UTailRudderCmd output; Pic_FlapCmd input
function [PrtAileronUpperCmd, PrtAileronLowerCmd, StbdAileronUpperCmd, StbdAileronLowerCmd,...
          PrtInbElevonCmd, StbdInbdElevonCmd, PrtOutElevonCmd, StbdOutdElevonCmd,...
          ElevatorUtailCmd, AftFlapCmd,...
          PylonRudderCmd, WingletRudderCmd, UTailRudderCmd]= fcn(Pic_AileronCmd, Pic_ElevatorCmd, Pic_RudderCmd, Pic_FlapCmd)
    
      % Mix ailerons as usual
      PrtAileronUpperCmd = Pic_AileronCmd;
      PrtAileronLowerCmd = Pic_AileronCmd;

      StbdAileronUpperCmd = Pic_AileronCmd;
      StbdAileronLowerCmd = Pic_AileronCmd;
      
      % Mix elevons as flaperons
      PrtInbElevonCmd   = min(Pic_AileronCmd + Pic_FlapCmd, 25);
      StbdInbdElevonCmd = min(-1*Pic_AileronCmd + Pic_FlapCmd, 25);
      
      PrtOutElevonCmd   = min(Pic_AileronCmd + Pic_FlapCmd, 25);
      StbdOutdElevonCmd = min(-1*Pic_AileronCmd + Pic_FlapCmd, 25);
      
      ElevatorUtailCmd = Pic_ElevatorCmd;
      AftFlapCmd = Pic_ElevatorCmd; 
      
      PylonRudderCmd   = Pic_RudderCmd;
      
      WingletRudderCmd = Pic_RudderCmd;
      
      UTailRudderCmd   = Pic_RudderCmd;      
end

== matlab function Lib_Piccolo/Control Allocation/M2 Flaperon and FTD/Surface Mixing Function ==
  data: Pic_AileronCmd input; PrtAileronUpperCmd output; Pic_ElevatorCmd input; PrtAileronLowerCmd output; StbdAileronUpperCmd output; StbdAileronLowerCmd output; PrtInbElevonCmd output; StbdInbdElevonCmd output; PrtOutElevonCmd output; StbdOutdElevonCmd output; ElevatorUtailCmd output; AftFlapCmd output; Pic_RudderCmd input; PylonRudderCmd output; WingletRudderCmd output; UTailRudderCmd output; Pic_FlapCmd input
function [PrtAileronUpperCmd, PrtAileronLowerCmd, StbdAileronUpperCmd, StbdAileronLowerCmd,...
          PrtInbElevonCmd, StbdInbdElevonCmd, PrtOutElevonCmd, StbdOutdElevonCmd,...
          ElevatorUtailCmd, AftFlapCmd,...
          PylonRudderCmd, WingletRudderCmd, UTailRudderCmd]= fcn(Pic_AileronCmd, Pic_ElevatorCmd, Pic_RudderCmd, Pic_FlapCmd)
    
      % Split Ailerons from flap command
      PrtAileronUpperCmd = max(-2 * Pic_FlapCmd + Pic_AileronCmd, -45);
      PrtAileronLowerCmd =  min(2 * Pic_FlapCmd + Pic_AileronCmd, 45);

      StbdAileronUpperCmd =  min(2 * Pic_FlapCmd + Pic_AileronCmd, 45);
      StbdAileronLowerCmd = max(-2 * Pic_FlapCmd + Pic_AileronCmd, -45);
      
      % Mix elevons as flaperons
      PrtInbElevonCmd   = min(Pic_AileronCmd + Pic_FlapCmd, 25);
      StbdInbdElevonCmd = min(-1*Pic_AileronCmd + Pic_FlapCmd, 25);
      
      PrtOutElevonCmd   = min(Pic_AileronCmd + Pic_FlapCmd, 25);
      StbdOutdElevonCmd = min(-1*Pic_AileronCmd + Pic_FlapCmd, 25);
      
      ElevatorUtailCmd = Pic_ElevatorCmd;
      AftFlapCmd = Pic_ElevatorCmd; 
      
      PylonRudderCmd   = Pic_RudderCmd;
      
      WingletRudderCmd = Pic_RudderCmd;
      
      UTailRudderCmd   = Pic_RudderCmd;      
end

== matlab function Lib_Piccolo/Pitch to Elevator/Reference Frame Conversion and Pitch Rate Limit Determination/AeroVsStruct_Limit/Load Factors (nMax,nMin) at current conditions  ==
  data: Q input; nMax output; Sw input; CL_Limit input; CL_Min input; m input; nMax_User input; nMin_User input; nMin output
function [nMax, nMin] = fcn(Q, Sw, CL_Limit,CL_Min, m, nMax_User, nMin_User)

nAero_Max=Sw*Q*CL_Limit/(m*9.81);
nAero_Min=Sw*Q*CL_Min/(m*9.81);
nMax=min(nMax_User,nAero_Max);
nMin=max(nMin_User, nAero_Min);
end

== matlab function Lib_Piccolo/Pitch to Elevator/Reference Frame Conversion and Pitch Rate Limit Determination/MATLAB Function ==
  data: PitchCmd_Euler input; PitchCmd_Body output; Pitch_Euler input; Roll_Euler input; Pitch_Body output; Scalar output; PitchRateCmd_Body output; PitchRateLimit_Max output; PitchRateLimit_Min output; V input; nMax input; nMin input; PitchRateMax_User input; nPrime_Max output; nPrime_Min output
function [PitchCmd_Body,Pitch_Body, Scalar, PitchRateCmd_Body, PitchRateLimit_Max, PitchRateLimit_Min,nPrime_Max,nPrime_Min] = fcn(PitchCmd_Euler, Pitch_Euler, Roll_Euler,V,nMax,nMin,PitchRateMax_User)
g=9.81;
cPhi=cos(Roll_Euler); % input should be in radian
if (0<=cPhi)&&(cPhi<0.5)
    cPhi=0.5;
elseif (0>cPhi)&&(cPhi>-0.5)
    cPhi=-0.5;
end
Scalar=1/cPhi;
PitchCmd_Body=PitchCmd_Euler*Scalar;
Pitch_Body=Pitch_Euler*Scalar;
% PitchRateCmd_Body=abs(sin(Roll_Euler))*g/(cPhi*V); 
PitchRateCmd_Body=(sin(Roll_Euler))^2*g/(cPhi*V); 
%PitchRateCmd_Body=sin(Roll_Euler)^2*g/(cPhi^2*V); 
% error in the documentation
% Wrong in the documentation !
% nPrime_Max=nMax*(1-g)*cos(Roll_Euler)*cos(Pitch_Euler); 
% nPrime_Min=nMin*(1-g)*cos(Roll_Euler)*cos(Pitch_Euler);
nPrime_Max=(nMax-1)*cos(Roll_Euler)*cos(Pitch_Euler);
nPrime_Min=(nMin-1)*cos(Roll_Euler)*cos(Pitch_Euler);

PitchRateLimit_Max=min(PitchRateCmd_Body+PitchRateMax_User, g*nPrime_Max/V);
PitchRateLimit_Min=max(PitchRateCmd_Body-PitchRateMax_User, g*nPrime_Min/V);

% PitchRateLimit_Max=PitchRateMax_User;
% PitchRateLimit_Min=-PitchRateMax_User;
% PitchRateLimit_Max=PitchRateCmd_Body+PitchRateMax_User;
% PitchRateLimit_Min=PitchRateCmd_Body-PitchRateMax_User;
end
